simulink model "native_mpc_corrected"  (R2024b)
settings: Solver=FixedStepAuto  StartTime=0.0  StopTime=10.0  FixedStep=T_sample  RelTol=1e-3
model workspace (MAT data in the model file):
  A_native_d = [0.999563282322  0.00979329297471; -0.0867353791957  0.958799856095]
  B_native_d = [0.000437012444077; 0.0867939220075]
  E_native_d = [4.93097995741e-05; 0.00979329297471]
  Q1 = 1
  Q2 = 0.002
  R1 = 0.01
  T_sample = 0.01
  a = -4.16238198247
  b = 8.86258812349
  c = -8.856610276
  f0 = 0.982785644836
settings Model: Creator=Arrow  LastModifiedBy=sk3547969879
settings OptimizationCC: ReuseModelBlockBuffer=off
settings RTWCC: GPUComputeCapability=3.5

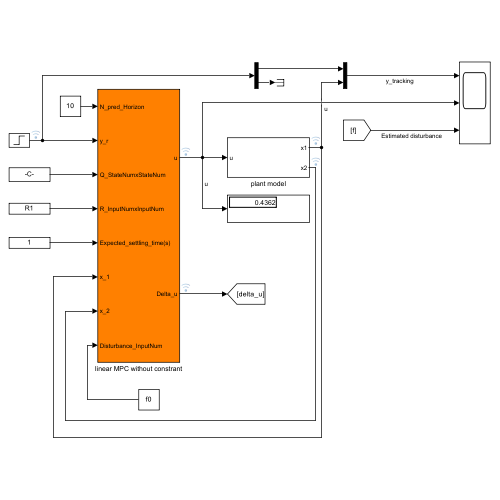
[thumbnail: Simulink's stored preview of the top-level diagram]
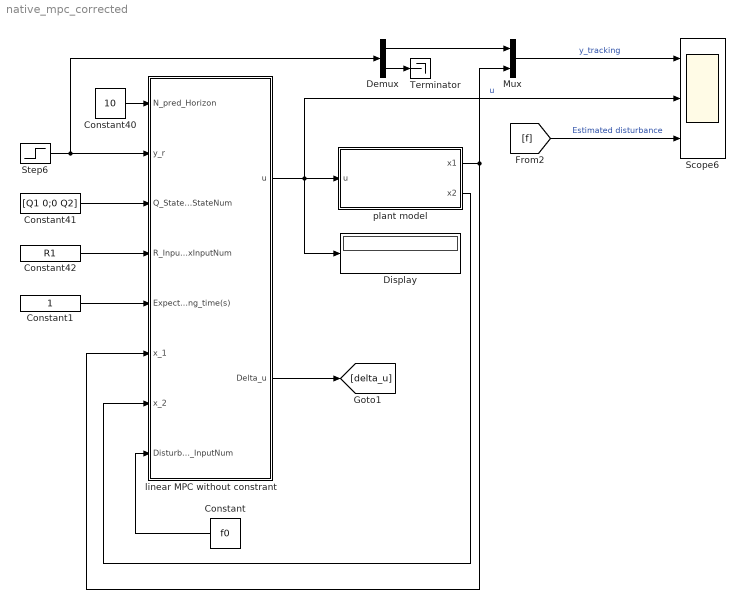
== system native_mpc_corrected ==
  Constant : Constant  Value=f0
  Constant1 : Constant
  Constant40 : Constant  Value=10
  Constant41 : Constant  Value=[Q1 0;0 Q2]
  Constant42 : Constant  Value=R1
  Demux : Demux  Outputs=2
  Display : Display
  Mux : Mux  Inputs=2
  Scope6 : Scope  NumInputPorts=3
  Step6 : Step  Time=5  Before=[0; 0]  After=[1; 0]  SampleTime=0
  Terminator : Terminator
  linear MPC without constrant : Subsystem
  plant model : Subsystem
  wires:
  Constant41/1 -> linear MPC without constrant/3(Q_StateNumxStateNum)
  linear MPC without constrant/1(u) -> Scope6/2, Display/1, plant model/1(u)  "u"
  Step6/1 -> Demux/1, linear MPC without constrant/2(y_r)
  Constant42/1 -> linear MPC without constrant/4(R_InputNumxInputNum)
  Mux/1 -> Scope6/1  "y_tracking"
  Constant40/1 -> linear MPC without constrant/1(N_pred_Horizon)
  plant model/2(x2) -> linear MPC without constrant/7(x_2)
  Constant1/1 -> linear MPC without constrant/5(Expected_settling_time(s))
  Demux/1 -> Mux/1
  Demux/2 -> Terminator/1
  plant model/1(x1) -> linear MPC without constrant/6(x_1), Mux/2
  linear MPC without constrant/2(Delta_u) -> [delta_u]
  Constant/1 -> linear MPC without constrant/8(Disturbance_InputNum)
  [f] -> Scope6/3  "Estimated disturbance"

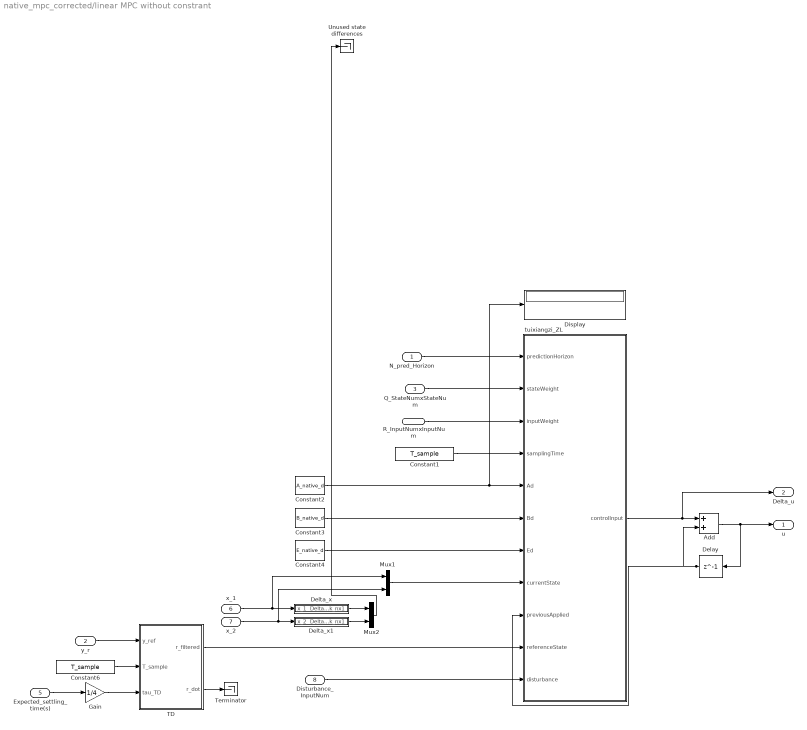
== system native_mpc_corrected/linear MPC without constrant ==
  N_pred_Horizon : Inport
  y_r : Inport  Port=2
  Q_StateNumxStateNum : Inport  Port=3
  R_InputNumxInputNum : Inport  Port=4
  Expected_settling_time(s) : Inport  Port=5
  x_1 : Inport  Port=6
  x_2 : Inport  Port=7
  Disturbance_InputNum : Inport  Port=8
  Add : Sum
  Constant1 : Constant  Value=T_sample
  Constant2 : Constant  Value=A_native_d
  Constant3 : Constant  Value=B_native_d
  Constant4 : Constant  Value=E_native_d
  Constant6 : Constant  Value=T_sample
  Delay : Delay  DelayLength=1
  Delta_x : Subsystem
  Delta_x1 : Subsystem
  Display : Display
  Gain : Gain  Gain=1/4
  Mux1 : Mux  Inputs=2
  Mux2 : Mux  Inputs=2
  TD : Subsystem
  Terminator : Terminator
  Unused state differences : Terminator
  tuixiangzi_ZL : MATLAB Function  TreatAsAtomicUnit=on
  u : Outport
  Delta_u : Outport  Port=2
  wires:
  tuixiangzi_ZL/1(controlInput) -> Delta_u/1, Add/1
  Constant1/1 -> tuixiangzi_ZL/4(samplingTime)
  Add/1 -> Delay/1, u/1
  Delay/1 -> Add/2, tuixiangzi_ZL/9(previousApplied)
  R_InputNumxInputNum/1 -> tuixiangzi_ZL/3(inputWeight)
  Mux1/1 -> tuixiangzi_ZL/8(currentState)
  x_1/1 -> Delta_x/1(x_1), Mux1/1
  x_2/1 -> Delta_x1/1(x_2), Mux1/2
  Delta_x/1(Delta_Xk_nx1) -> Mux2/1
  Delta_x1/1(Delta_Xk_nx1) -> Mux2/2
  Disturbance_InputNum/1 -> tuixiangzi_ZL/11(disturbance)
  Q_StateNumxStateNum/1 -> tuixiangzi_ZL/2(stateWeight)
  N_pred_Horizon/1 -> tuixiangzi_ZL/1(predictionHorizon)
  Constant2/1 -> Display/1, tuixiangzi_ZL/5(Ad)
  Constant3/1 -> tuixiangzi_ZL/6(Bd)
  Constant4/1 -> tuixiangzi_ZL/7(Ed)
  Constant6/1 -> TD/2(T_sample)
  TD/2(r_dot) -> Terminator/1
  Gain/1 -> TD/3(tau_TD)
  Expected_settling_time(s)/1 -> Gain/1
  y_r/1 -> TD/1(y_ref)
  TD/1(r_filtered) -> tuixiangzi_ZL/10(referenceState)
  Mux2/1 -> Unused state differences/1

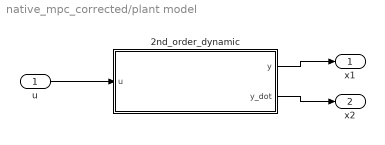
== system native_mpc_corrected/plant model ==
  u : Inport
  2nd_order_dynamic : Subsystem
  x1 : Outport
  x2 : Outport  Port=2
  wires:
  2nd_order_dynamic/2(y_dot) -> x2/1
  u/1 -> 2nd_order_dynamic/1(u)
  2nd_order_dynamic/1(y) -> x1/1

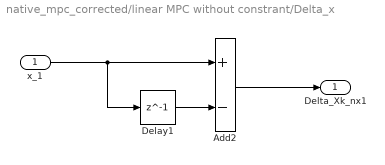
== system native_mpc_corrected/linear MPC without constrant/Delta_x ==
  x_1 : Inport
  Add2 : Sum  Inputs=+-
  Delay1 : Delay  DelayLength=1  InitialCondition=0
  Delta_Xk_nx1 : Outport
  wires:
  Delay1/1 -> Add2/2
  x_1/1 -> Delay1/1, Add2/1
  Add2/1 -> Delta_Xk_nx1/1

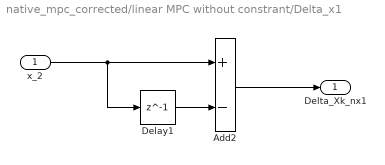
== system native_mpc_corrected/linear MPC without constrant/Delta_x1 ==
  x_2 : Inport
  Add2 : Sum  Inputs=+-
  Delay1 : Delay  DelayLength=1  InitialCondition=0
  Delta_Xk_nx1 : Outport
  wires:
  Add2/1 -> Delta_Xk_nx1/1
  x_2/1 -> Add2/1, Delay1/1
  Delay1/1 -> Add2/2

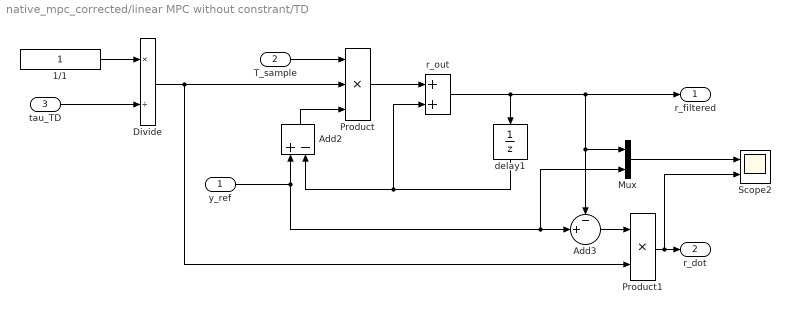
== system native_mpc_corrected/linear MPC without constrant/TD ==
  y_ref : Inport
  T_sample : Inport  Port=2
  tau_TD : Inport  Port=3
  1/1 : Constant
  Add2 : Sum  Inputs=+-
  Add3 : Sum  Inputs=-+|
  Divide : Product  Inputs=*/
  Mux : Mux  Inputs=2
  Product : Product  Inputs=3  RndMeth=Zero
  Product1 : Product  RndMeth=Zero
  Scope2 : Scope  NumInputPorts=2
  delay1 : UnitDelay  SampleTime=-1  HasFrameUpgradeWarning=on
  r_out : Sum
  r_filtered : Outport  VectorParamsAs1DForOutWhenUnconnected=off
  r_dot : Outport  Port=2  VectorParamsAs1DForOutWhenUnconnected=off
  wires:
  T_sample/1 -> Product/1
  Divide/1 -> Product1/2, Product/2
  Add3/1 -> Product1/1
  r_out/1 -> r_filtered/1, Mux/1, Add3/1, delay1/1
  Add2/1 -> Product/3
  Product1/1 -> Scope2/2, r_dot/1
  delay1/1 -> r_out/2, Add2/2
  y_ref/1 -> Mux/2, Add3/2, Add2/1
  Product/1 -> r_out/1
  Mux/1 -> Scope2/1
  1/1/1 -> Divide/1
  tau_TD/1 -> Divide/2

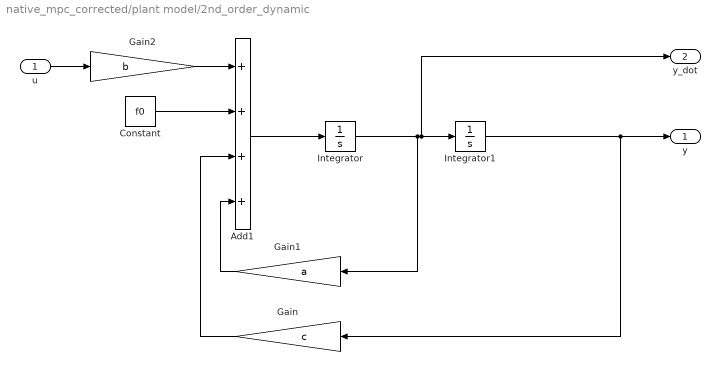
== system native_mpc_corrected/plant model/2nd_order_dynamic ==
  u : Inport
  Add1 : Sum  Inputs=++++
  Constant : Constant  Value=f0
  Gain : Gain  Gain=c
  Gain1 : Gain  Gain=a
  Gain2 : Gain  Gain=b
  Integrator : Integrator
  Integrator1 : Integrator
  y : Outport
  y_dot : Outport  Port=2
  wires:
  Add1/1 -> Integrator/1
  Gain/1 -> Add1/3
  u/1 -> Gain2/1
  Integrator/1 -> Gain1/1, y_dot/1, Integrator1/1
  Integrator1/1 -> Gain/1, y/1
  Gain2/1 -> Add1/1
  Gain1/1 -> Add1/4
  Constant/1 -> Add1/2

== matlab function native_mpc_corrected/linear MPC without constrant/tuixiangzi_ZL ==
  settings: updateMethod=DISCRETE  sampleTime=T_sample
  data: predictionHorizon input; controlInput output size=1; stateWeight input; inputWeight input; samplingTime input; Ad input; Bd input; Ed input; currentState input; previousApplied input; referenceState input; disturbance input
function controlInput = MPC_bounded(predictionHorizon,stateWeight,inputWeight,samplingTime,Ad,Bd,Ed,currentState,previousApplied,referenceState,disturbance)
%#codegen
% Input 9 carries the previous applied command. Ports 5 to 7 carry ZOH matrices.
assert(predictionHorizon==10);
[u,status] = native_mpc_step(Ad,Bd,Ed,currentState,previousApplied,referenceState,disturbance,stateWeight,inputWeight,samplingTime);
assert(status==1);
controlInput=u-previousApplied;
end
